simulink model "cp6_ej1_zn"  (R2026a)
settings: Solver=VariableStepAuto  StopTime=20  MaxStep=0.002
libraries: slpidlib x1
settings Model: Creator=benja  LastModifiedBy=benja

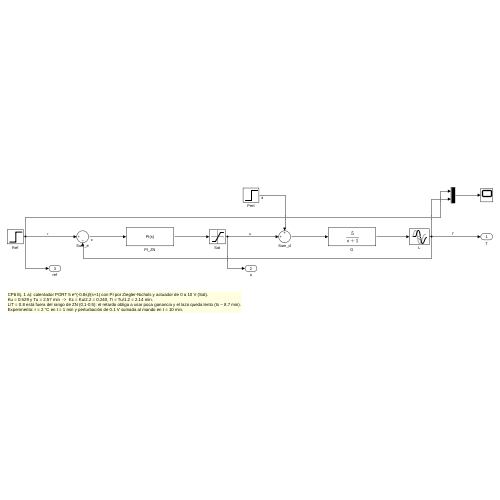
[thumbnail: Simulink's stored preview of the top-level diagram]
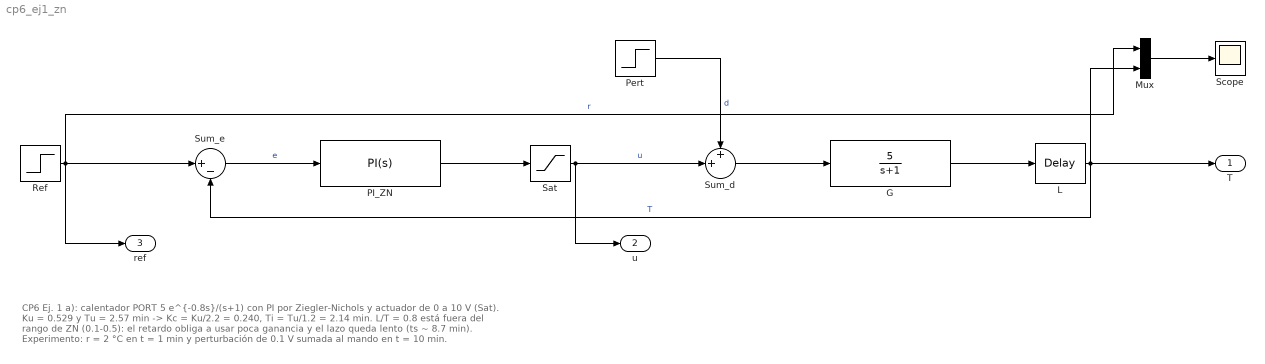
== system cp6_ej1_zn ==
  note: CP6 Ej. 1 a): calentador PORT 5 e^{-0.8s}/(s+1) con PI por Ziegler-Nichols y actuador de 0 a 10 V (Sat).
      | Ku = 0.529 y Tu = 2.57 min  ->  Kc = Ku/2.2 = 0.240, Ti = Tu/1.2 = 2.14 min.
      | L/T = 0.8 está fuera del rango de ZN (0.1-0.5): el retardo obliga a usar poca ganancia y el lazo queda lento (ts ~ 8.7 min).
      | Experimento: r = 2 °C en t = 1 min y perturbación de 0.1 V sumada al mando en t = 10 min.
  G : TransferFcn  Numerator=5  Denominator=[1 1]
  L : TransportDelay  DelayTime=0.8
  Mux : Mux  Inputs=2
  PI_ZN : slpidlib/PID Controller  Controller=PI  Form=Parallel  TimeDomain=Continuous-time  UseExternalTs=off  SampleTime=-1  IntegratorMethod=Forward Euler  FilterMethod=Forward Euler  ControllerParametersSource=internal  P=0.2404  I=0.1124  UseKiTs=off  D=0  UseExternalDerivativeSource=off  N=100  UseFilter=on  TunerSelectOption=Transfer Function Based (PID Tuner App)  InitialConditionSource=internal  InitialConditionForIntegrator=0  InitialConditionForFilter=0  DifferentiatorICPrevScaledInput=0  ExternalReset=none  TrackingMode=off  Kt=1  LimitOutput=off  SatLimitsSource=internal  UpperSaturationLimit=inf  LowerSaturationLimit=-inf  LinearizeAsGain=on  AntiWindupMode=none  Kb=1  LimitIntegrator=off  UpperIntegratorSaturationLimit=inf  LowerIntegratorSaturationLimit=-inf  POutMin=[]  POutMax=[]  IOutMin=[]  IOutMax=[]  DOutMin=[]  DOutMax=[]  NOutMin=[]  NOutMax=[]  SumOutMin=[]  SumOutMax=[]  SaturationOutMin=[]  SaturationOutMax=[]  PParamMin=[]  PParamMax=[]  IParamMin=[]  IParamMax=[]  DParamMin=[]  DParamMax=[]  NParamMin=[]  NParamMax=[]  KbParamMin=[]  KbParamMax=[]  KtParamMin=[]  KtParamMax=[]  KbOutMin=[]  KbOutMax=[]  KtOutMin=[]  KtOutMax=[]  IntegratorOutMin=[]  IntegratorOutMax=[]  FilterOutMin=[]  FilterOutMax=[]  SumI1OutMin=[]  SumI1OutMax=[]  SumI2OutMin=[]  SumI2OutMax=[]  SumI3OutMin=[]  SumI3OutMax=[]  SumI4OutMin=[]  SumI4OutMax=[]  SumDOutMin=[]  SumDOutMax=[]  DifferentiatorOutMin=[]  DifferentiatorOutMax=[]  FilterDiffOutCoefMin=[]  FilterDiffOutCoefMax=[]  ReciprocalOutMin=[]  ReciprocalOutMax=[]  SumDenOutMin=[]  SumDenOutMax=[]  SumNumOutMin=[]  SumNumOutMax=[]  DivideOutMin=[]  DivideOutMax=[]  UdiffTsProdOutMin=[]  UdiffTsProdOutMax=[]  NTsProdOutMin=[]  NTsProdOutMax=[]  UintegralTsProdOutMin=[]  UintegralTsProdOutMax=[]  UngainTsProdOutMin=[]  UngainTsProdOutMax=[]  ClampingZeroOutDataTypeStr=Inherit: Inherit via back propagation  ClampingZeroOutMin=[]  ClampingZeroOutMax=[]  FilterDenConstantOutDataTypeStr=Inherit: Inherit via back propagation  FilterDenConstantOutMin=[]  FilterDenConstantOutMax=[]  PCopyOutDataTypeStr=Inherit: Inherit via back propagation  PCopyOutMin=[]  PCopyOutMax=[]  NCopyOutDataTypeStr=Inherit: Inherit via back propagation  NCopyOutMin=[]  NCopyOutMax=[]  IntegratorContinuousStateAttributes=''  IntegratorStateMustResolveToSignalObject=off  IntegratorRTWStateStorageClass=Auto  FilterContinuousStateAttributes=''  FilterStateMustResolveToSignalObject=off  FilterRTWStateStorageClass=Auto  ParallelPVariant=InternalParameters  IdealPVariant=Disabled  IVariant=InternalParameters  DVariant=Disabled  IntegratorVariant=Continuous  SatVariant=Disabled  AWVariant=Passthrough  PCopyVariant=Disabled  TRVariant=Disabled  FdbkBlocksVariant=Forward  IdealPFdbkVariant=Disabled  SatFdbkVariant=Disabled  DerivativeFilterVariant=Disabled  NVariant=Disabled  NCopyVariant=Disabled_SignalSpec  FilterICVariant=Disabled  IntegratorICVariant=InternalICs  ExternalResetVariant=Disabled  TRSumVariant=Passthrough  SumFdbkVariant=Disabled  SumVariant=Sum_PI  TsampFilterVariant=InternalTs  TsampNgainVariant=Passthrough  TsampIntegralVariant=Disabled_SignalSpec  ExternalSaturationOutDataTypeStr=Inherit: Same as second input  DerivativeSourceVariant=Disabled  PreIntVariant=InternalPreInt
  Pert : Step  Time=10  FinalValue=0.1  SampleTime=0
  Ref : Step  FinalValue=2  SampleTime=0
  Sat : Saturate  UpperLimit=10  LowerLimit=0
  Scope : Scope
  Sum_d : Sum  Inputs=++|
  Sum_e : Sum  Inputs=|+-
  T : Outport
  u : Outport  Port=2
  ref : Outport  Port=3
  wires:
  Ref/1 -> Sum_e/1, ref/1, Mux/1  "r"
  Sum_e/1 -> PI_ZN/1  "e"
  PI_ZN/1 -> Sat/1
  Sat/1 -> Sum_d/2, u/1  "u"
  Pert/1 -> Sum_d/1  "d"
  Sum_d/1 -> G/1
  G/1 -> L/1
  L/1 -> T/1, Sum_e/2, Mux/2  "T"
  Mux/1 -> Scope/1
